simulink model "EV_BMS"  (R2026a)
settings: Solver=VariableStepAuto  StopTime=100
undefined symbols (not defined in the file): battery_builder_rtmsupport, gcbh
libraries: simulink x27, fl_lib x3, nesl_utility x2, EV_BMS_Thermal_lib x1, simulink_extras x1

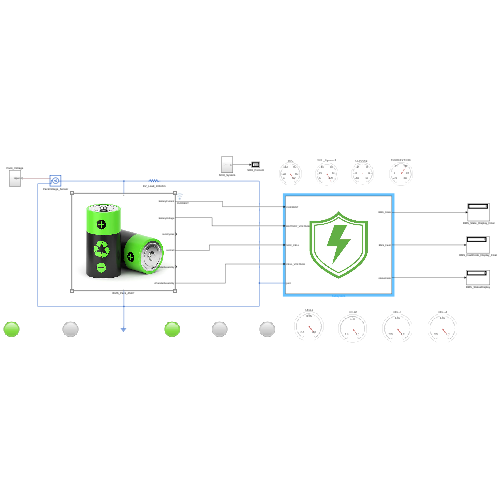
[thumbnail: Simulink's stored preview of the top-level diagram]
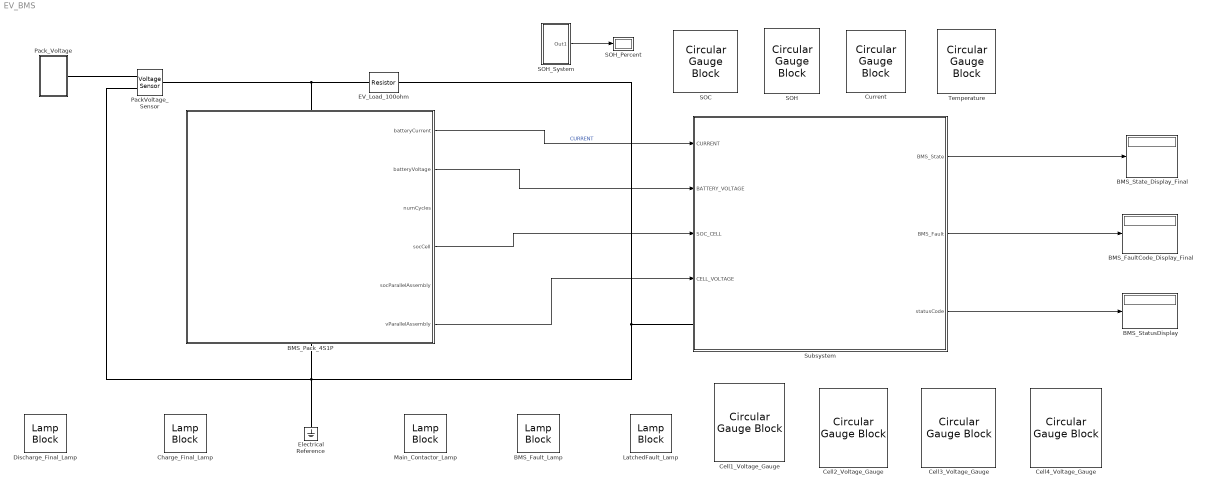
== system EV_BMS ==
  BMS_FaultCode_Display_Final : Display
  BMS_Fault_Lamp : LampBlock  LabelPosition=Hide  DefaultColor=[192.0, 192.0, 192.0]
  BMS_Pack_4S1P : Subsystem  LoadFcn=battery_builder_rtmsupport('loadfcn',gcbh);
      settings: CopyFcn=battery_builder_rtmsupport('copyfcn',gcbh);  PreCopyFcn=battery_builder_rtmsupport('precopyfcn',gcbh);  PreDeleteFcn=battery_builder_rtmsupport('predeletefcn',gcbh);  PortSchema="{\"entries\":[{\"content\":{\"sides\":[{\"content\":{\"connectorIds\":[\"LConn1\"]},\"type\":\"ConnectorPlacement.EquallySpacedRectSide\",\"uuid\":\"f9609fd6-83a3-4776-8a05-b3fc995cf9f2\"},{\"content\":{\"connectorIds\":[\"RConn1\"],\"side\":\"RIGHT\"},\"type\":\"ConnectorPlacement.EquallySpacedRectSide\",\"uuid\":\"cb6b546a-39c6-443d-8083-a29f501cd994\"},{\"content\":{\"side\":\"TOP\"},\"type\":\"ConnectorPlacement.EquallySpacedRectSide\",\"uuid\":\"97627d3a-e8ea-48cc-9b43-c4f6fa748c18\"},{\"content\":{\"connectorIds\":[\"Out1\",\"Out2\",\"Out3\",\"Out4\",\"Out5\",\"Out6\"],\"side\":\"BOTTOM\"},\"type\":\"ConnectorPlacement.EquallySpacedRectSide\",\"uuid\":\"a53582b5-eaea-45ee-b7fe-337964f2a653\"}]},\"type\":\"ConnectorPlacement.EquallySpacedConnector\",\"uuid\":\"342c31db-417c-4e7c-9c09-9d8ea7b34008\"}],\"packageUris\":[\"http://schema.mathworks.com/mf0/Connector/R2020b\"],\"version\":\"1.0\"}"
      mask Display: image('WhatsApp Image 2026-08-24 at 3.32.36 PM (1).jpeg');
  BMS_State_Display_Final : Display
  BMS_StatusDisplay : Display
  Cell1_Voltage_Gauge : CircularGaugeBlock  ScaleMin=2.5  ScaleMax=4.2  FontColor=[0.0, 0.0, 0.0]
  Cell2_Voltage_Gauge : CircularGaugeBlock  ScaleMin=2.5  ScaleMax=4.2  FontColor=[0.0, 0.0, 0.0]
  Cell3_Voltage_Gauge : CircularGaugeBlock  ScaleMin=2.5  ScaleMax=4.2  FontColor=[0.0, 0.0, 0.0]
  Cell4_Voltage_Gauge : CircularGaugeBlock  ScaleMin=2.5  ScaleMax=4.2  FontColor=[0.0, 0.0, 0.0]
  Charge_Final_Lamp : LampBlock  LabelPosition=Hide  DefaultColor=[192.0, 192.0, 192.0]
  Current : CircularGaugeBlock  ScaleMin=-10  ScaleMax=10  FontColor=[0.0, 0.0, 0.0]
  Discharge_Final_Lamp : LampBlock  LabelPosition=Hide  DefaultColor=[192.0, 192.0, 192.0]
  EV_Load_100ohm : fl_lib/Electrical/Electrical Elements/Resistor  R=10 Ohm  i_specify=off  i_priority=None  i=0 A  i_nominal_specify=off  i_nominal_value=1  i_nominal_unit=A  v_specify=off  v_priority=None  v=0 V  v_nominal_specify=off  v_nominal_value=1  v_nominal_unit=V
  Electrical Reference : fl_lib/Electrical/Electrical Elements/Electrical Reference
  LatchedFault_Lamp : LampBlock  LabelPosition=Hide  DefaultColor=[192.0, 192.0, 192.0]
  Main_Contactor_Lamp : LampBlock  LabelPosition=Hide  DefaultColor=[192.0, 192.0, 192.0]
  PackVoltage_Sensor : fl_lib/Electrical/Electrical Sensors/Voltage Sensor
  Pack_Voltage : Subsystem
  SOC : CircularGaugeBlock  FontColor=[0.0, 0.0, 0.0]
  SOH : CircularGaugeBlock  FontColor=[0.0, 0.0, 0.0]
  SOH_Percent : Display
  SOH_System : Subsystem
  Subsystem : Subsystem
      mask Display: image('WhatsApp Image 2026-08-24 at 3.45.53 PM.jpeg');
  Temperature : CircularGaugeBlock  ScaleMin=-20  ScaleMax=60  FontColor=[0.0, 0.0, 0.0]
  wires:
  SOH_System/1(Out1) -> SOH_Percent/1
  BMS_Pack_4S1P/1(batteryCurrent) -> Subsystem/1(CURRENT)  "CURRENT"
  BMS_Pack_4S1P/2(batteryVoltage) -> Subsystem/2(BATTERY_VOLTAGE)
  BMS_Pack_4S1P/4(socCell) -> Subsystem/3(SOC_CELL)
  BMS_Pack_4S1P/6(vParallelAssembly) -> Subsystem/4(CELL_VOLTAGE)
  Subsystem/1(BMS_State) -> BMS_State_Display_Final/1
  Subsystem/2(BMS_Fault) -> BMS_FaultCode_Display_Final/1
  Subsystem/3(statusCode) -> BMS_StatusDisplay/1
  connections:
  PackVoltage_Sensor/RConn2 -- Subsystem/LConn1 -- EV_Load_100ohm/RConn1 -- BMS_Pack_4S1P/RConn1 -- Electrical Reference/LConn1
  EV_Load_100ohm/LConn1 -- BMS_Pack_4S1P/LConn1 -- PackVoltage_Sensor/LConn1
  Pack_Voltage/LConn1 -- PackVoltage_Sensor/RConn1

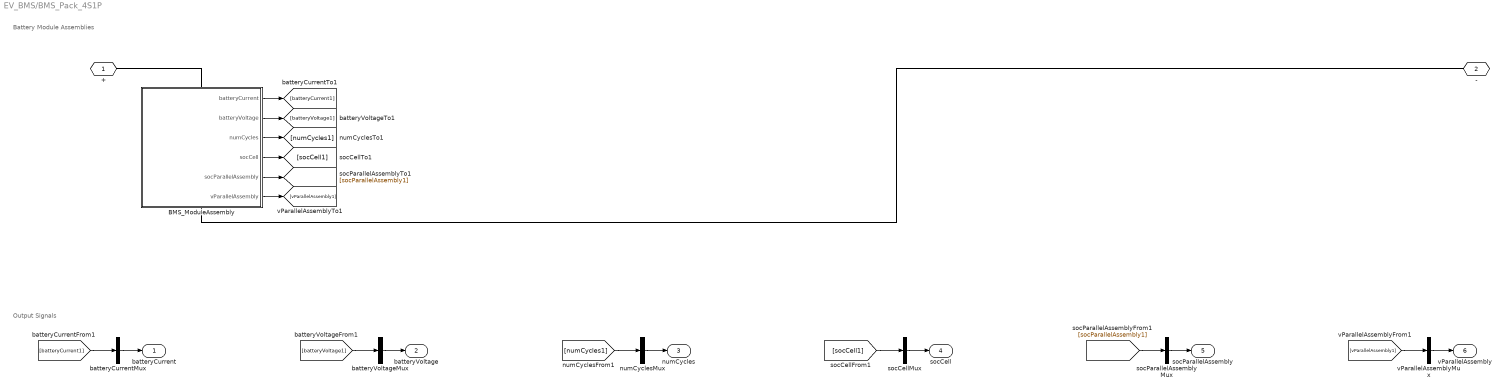
== system EV_BMS/BMS_Pack_4S1P ==
  note: Battery Module Assemblies
  note: Output Signals
  BMS_ModuleAssembly : Subsystem  LoadFcn=battery_builder_rtmsupport('loadfcn',gcbh);
      settings: CopyFcn=battery_builder_rtmsupport('copyfcn',gcbh);  PreCopyFcn=battery_builder_rtmsupport('precopyfcn',gcbh);  PreDeleteFcn=battery_builder_rtmsupport('predeletefcn',gcbh);  PortSchema="{\"entries\":[{\"content\":{\"sides\":[{\"content\":{\"connectorIds\":[\"LConn1\"]},\"type\":\"ConnectorPlacement.EquallySpacedRectSide\",\"uuid\":\"f9609fd6-83a3-4776-8a05-b3fc995cf9f2\"},{\"content\":{\"connectorIds\":[\"RConn1\"],\"side\":\"RIGHT\"},\"type\":\"ConnectorPlacement.EquallySpacedRectSide\",\"uuid\":\"cb6b546a-39c6-443d-8083-a29f501cd994\"},{\"content\":{\"side\":\"TOP\"},\"type\":\"ConnectorPlacement.EquallySpacedRectSide\",\"uuid\":\"97627d3a-e8ea-48cc-9b43-c4f6fa748c18\"},{\"content\":{\"connectorIds\":[\"Out1\",\"Out2\",\"Out3\",\"Out4\",\"Out5\",\"Out6\"],\"side\":\"BOTTOM\"},\"type\":\"ConnectorPlacement.EquallySpacedRectSide\",\"uuid\":\"d854d543-752b-4c93-bd7e-44390da1a379\"}]},\"type\":\"ConnectorPlacement.EquallySpacedConnector\",\"uuid\":\"342c31db-417c-4e7c-9c09-9d8ea7b34008\"}],\"packageUris\":[\"http://schema.mathworks.com/mf0/Connector/R2020b\"],\"version\":\"1.0\"}"
      mask Display: image('moduleAssembly_1.JPG');
  batteryCurrentMux : Mux  Inputs=1
  batteryVoltageMux : Mux  Inputs=1
  numCyclesMux : Mux  Inputs=1
  socCellMux : Mux  Inputs=1
  socParallelAssemblyMux : Mux  Inputs=1
  vParallelAssemblyMux : Mux  Inputs=1
  + : PMIOPort  Side=Left
  - : PMIOPort  Port=2  Side=Right
  batteryCurrent : Outport
  batteryVoltage : Outport  Port=2
  numCycles : Outport  Port=3
  socCell : Outport  Port=4
  socParallelAssembly : Outport  Port=5
  vParallelAssembly : Outport  Port=6
  wires:
  BMS_ModuleAssembly/1(batteryCurrent) -> [batteryCurrent1]
  batteryCurrentMux/1 -> batteryCurrent/1
  [batteryCurrent1] -> batteryCurrentMux/1
  BMS_ModuleAssembly/2(batteryVoltage) -> [batteryVoltage1]
  batteryVoltageMux/1 -> batteryVoltage/1
  [batteryVoltage1] -> batteryVoltageMux/1
  BMS_ModuleAssembly/3(numCycles) -> [numCycles1]
  numCyclesMux/1 -> numCycles/1
  [numCycles1] -> numCyclesMux/1
  BMS_ModuleAssembly/4(socCell) -> [socCell1]
  socCellMux/1 -> socCell/1
  [socCell1] -> socCellMux/1
  BMS_ModuleAssembly/5(socParallelAssembly) -> [socParallelAssembly1]
  socParallelAssemblyMux/1 -> socParallelAssembly/1
  [socParallelAssembly1] -> socParallelAssemblyMux/1
  BMS_ModuleAssembly/6(vParallelAssembly) -> [vParallelAssembly1]
  vParallelAssemblyMux/1 -> vParallelAssembly/1
  [vParallelAssembly1] -> vParallelAssemblyMux/1
  connections:
  BMS_ModuleAssembly/LConn1 -- +/RConn1
  BMS_ModuleAssembly/RConn1 -- -/RConn1

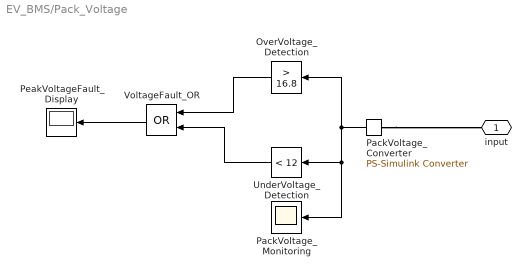
== system EV_BMS/Pack_Voltage ==
  " PackVoltage_Converter" : nesl_utility/PS-Simulink Converter  PhysicalDomain=network_engine_domain  SubClassName=ps_output  LeftPortType=input  RightPortType=output  PseudoPeriodic=off  Frequencies=[]  VectorFormat=inherit  Unit=inherit  AffineConversion=off
  OverVoltage_Detection : simulink/Logic and Bit Operations/Compare To Constant  relop=>  const=16.8  OutDataTypeStr=boolean
  PackVoltage_Monitoring : Scope
      settings: ActiveDisplayYMinimum=16.664557176862598  ActiveDisplayYMaximum=16.709356827128964
  PeakVoltageFault_Display : Display
  UnderVoltage_Detection : simulink/Logic and Bit Operations/Compare To Constant  relop=<  const=12  OutDataTypeStr=boolean
  VoltageFault_OR : Logic  Operator=OR  AllPortsSameDT=off  OutDataTypeStr=boolean
  input : PMIOPort  Side=Left
  wires:
  " PackVoltage_Converter"/1 -> PackVoltage_Monitoring/1, UnderVoltage_Detection/1, OverVoltage_Detection/1
  VoltageFault_OR/1 -> PeakVoltageFault_Display/1
  OverVoltage_Detection/1 -> VoltageFault_OR/1
  UnderVoltage_Detection/1 -> VoltageFault_OR/2
  connections:
  " PackVoltage_Converter"/LConn1 -- input/RConn1

== system EV_BMS/SOH_System ==
  Available_Capacity : Constant  Value=10
  Divide : Product  Inputs=*/
  Gain1 : Gain  Gain=100
  Rated_Capacity : Constant  Value=10
  Out1 : Outport
  wires:
  Rated_Capacity/1 -> Divide/2
  Available_Capacity/1 -> Divide/1
  Divide/1 -> Gain1/1
  Gain1/1 -> Out1/1

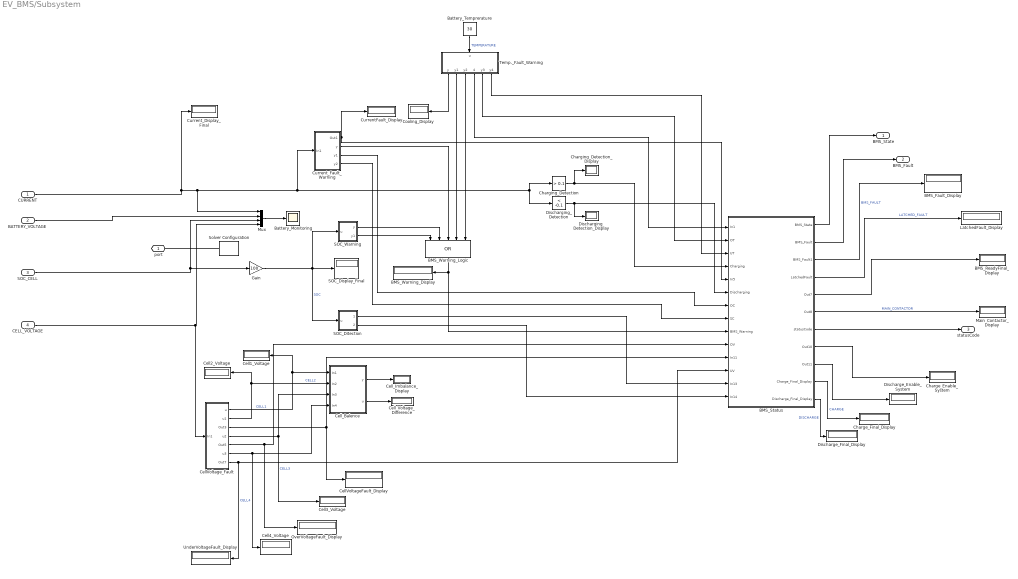
== system EV_BMS/Subsystem ==
  CURRENT : Inport
  BATTERY_VOLTAGE : Inport  Port=2
  SOC_CELL : Inport  Port=3
  CELL_VOLTAGE : Inport  Port=4
  BMS_Fault_Display : Display
  BMS_ReadyFinal_Display : Display
  BMS_Status : Subsystem
  BMS_Warning_Display : Display
  BMS_Warning_Logic : Logic  Operator=OR  Inputs=5  AllPortsSameDT=off  OutDataTypeStr=boolean
  Battery_Monitoring : Scope
      settings: ActiveDisplayYMinimum=-3.3250860487135681  ActiveDisplayYMaximum=5.1404092347440722
  Battery_Temprerature : Constant  Value=30
  Cell1_Voltage : Display
  Cell2_Voltage : Display
  Cell3_Voltage : Display
  Cell4_Voltage : Display
  CellVoltageFault_Display : Display
  CellVoltage_Fault : Subsystem
  Cell_Balence : Subsystem
  Cell_Imbalance_Display : Display
  Cell_Voltage_Difference : Display
  Charge_Enable_System : Display
  Charge_Final_Display : Display
  Charging_Detection : simulink/Logic and Bit Operations/Compare To Constant  relop=>  const=0.1  OutDataTypeStr=boolean
  Charging_Detection_Display : Display
  Cooling_Display : Display
  CurrentFault_Display : Display
  Current_Display_Final : Display
  Current_Fault_Warning : Subsystem
  Discharge_Enable_System : Display
  Discharge_Final_Display : Display
  Discharging_Detection : simulink/Logic and Bit Operations/Compare To Constant  relop=<  const=-0.1  OutDataTypeStr=boolean
  Discharging_Detection_Display : Display
  Gain : Gain  Gain=100
  LatchedFault_Display : Display
  Main_Contactor_Display : Display
  Mux : Mux
  OverVoltageFault_Display : Display
  SOC_Display_Final : Display
  SOC_Ditection : Subsystem
  SOC_Warning : Subsystem
  Solver Configuration : nesl_utility/Solver Configuration  PhysicalDomain=network_engine_domain  SubClassName=solver  LeftPortType=input  RightPortType=generic  Tones=[]  Harmonics=[]  SimulateNoise=off  Profile=off  UseLocalSampling=off  EnableSwitchedLinearOptims=on  FrequencyDomain=off  UseCCode=off  RelTol=0.001  AbsTol=0.001  MinStep=1e-09  ToWorkspace=off  RevertToSquareIcSolve=off  NumHomotopyIterations=100  PhasorMode=off  PhasorModeNumHarmonics=1  ConsistencySolver=NEWTON_XTOL_AFTER_FTOL  CanonicalOrdering=CANONICAL  OptimizeIntermediates=OPTIMIZED  IndexReductionMethod=DerivativeReplacement  DoDC=off  ResidualTolerance=1e-09  ConsistencyTolSource=GLOBAL  ConsistencyAbsTol=0.001  ConsistencyRelTol=0.001  ConsistencyTolFactor=0.001  UseLocalSolver=off  LocalSolverChoice=NE_BACKWARD_EULER_ADVANCER  ResolveIndetEquations=on  FunctionEvalNumThread=1  LocalSolverSampleTime=0.001  DoFixedCost=off  MaxNonlinIter=3  MaxModeIter=2  ComputeImpulses=off  ImpulseIterations=2  LinearAlgebra=auto  LinearAlgebraNumThread=0  EquationFormulation=NE_TIME_EF  DelaysMemoryBudget=1024  AutomaticFiltering=on  FilteringTimeConstant=0.001  PartitionStorageMethod=AS_NEEDED  PartitionMemoryBudget=1024  PartitionMethod=ROBUST  MultibodyUseLocalSolver=off  MultibodyLocalSolverChoice=ODE1  MultibodyLocalSolverSampleTime=0.001
  Temp._Fault_Warning : Subsystem
  UnderVoltageFault_Display : Display
  port : PMIOPort  Side=Left
  BMS_State : Outport
  BMS_Fault : Outport  Port=2
  statusCode : Outport  Port=3
  wires:
  BMS_Status/6(Out8) -> Main_Contactor_Display/1  "MAIN_CONTACTOR"
  Cell_Balence/2(u) -> Cell_Voltage_Difference/1
  BMS_Status/10(Charge_Final_Display) -> Charge_Final_Display/1  "CHARGE"
  BMS_Status/4(LatchedFault) -> LatchedFault_Display/1  "LATCHED_FAULT"
  SOC_Warning/1(y) -> BMS_Warning_Logic/2
  Cell_Balence/1(y) -> Cell_Imbalance_Display/1
  Temp._Fault_Warning/4(Out4) -> BMS_Status/1(In1)
  BMS_Status/3(BMS_Fault1) -> BMS_Fault_Display/1  "BMS_FAULT"
  CellVoltage_Fault/1(u) -> Cell1_Voltage/1, Cell_Balence/1(In1)  "CELL1"
  Current_Fault_Warning/2(y) -> BMS_Warning_Logic/3
  Temp._Fault_Warning/1(y) -> Cooling_Display/1
  SOC_Ditection/1(Out1) -> BMS_Status/13(In13)
  BMS_Status/11(Discharge_Final_Display) -> Discharge_Final_Display/1  "DISCHARGE"
  Temp._Fault_Warning/5(y3) -> BMS_Status/2(OT)
  CellVoltage_Fault/6(u3) -> Cell4_Voltage/1, Cell_Balence/4(In4)  "CELL4"
  Battery_Temprerature/1 -> Temp._Fault_Warning/1(u)  "TEMPERATURE"
  Temp._Fault_Warning/2(y1) -> BMS_Warning_Logic/4
  SOC_Ditection/2(Out2) -> BMS_Status/14(In14)
  Current_Fault_Warning/3(y1) -> BMS_Status/7(OC)
  BMS_Status/2(BMS_Fault) -> BMS_Fault/1
  CellVoltage_Fault/4(u2) -> Cell3_Voltage/1, Cell_Balence/3(In3)  "CELL3"
  Charging_Detection/1 -> Charging_Detection_Display/1, BMS_Status/4(Charging)
  Temp._Fault_Warning/6(y4) -> BMS_Status/3(UT)
  CELL_VOLTAGE/1 -> Mux/4, CellVoltage_Fault/1(In1)
  BMS_Status/5(Out7) -> BMS_ReadyFinal_Display/1
  CURRENT/1 -> Current_Display_Final/1, Charging_Detection/1, Discharging_Detection/1, Current_Fault_Warning/1(In1), Mux/1
  CellVoltage_Fault/3(Out3) -> BMS_Status/11(In11), CellVoltageFault_Display/1
  BMS_Status/1(BMS_State) -> BMS_State/1
  BMS_Warning_Logic/1 -> BMS_Status/9(BMS_Warning), BMS_Warning_Display/1
  Gain/1 -> SOC_Warning/1(u), SOC_Display_Final/1, SOC_Ditection/1(u)  "SOC"
  BATTERY_VOLTAGE/1 -> Mux/2
  BMS_Status/7(statusCode) -> statusCode/1
  Current_Fault_Warning/1(Out1) -> BMS_Status/5(In5), CurrentFault_Display/1
  SOC_CELL/1 -> Mux/3, Gain/1
  Temp._Fault_Warning/3(y2) -> BMS_Warning_Logic/5
  SOC_Warning/2(y1) -> BMS_Warning_Logic/1
  CellVoltage_Fault/5(Out5) -> BMS_Status/10(OV), OverVoltageFault_Display/1
  Current_Fault_Warning/4(y2) -> BMS_Status/8(SC)
  CellVoltage_Fault/7(Out7) -> UnderVoltageFault_Display/1, BMS_Status/12(UV)
  CellVoltage_Fault/2(u1) -> Cell_Balence/2(In2), Cell2_Voltage/1  "CELL2"
  BMS_Status/8(Out10) -> Charge_Enable_System/1
  Mux/1 -> Battery_Monitoring/1
  Discharging_Detection/1 -> BMS_Status/6(Discharging), Discharging_Detection_Display/1
  BMS_Status/9(Out11) -> Discharge_Enable_System/1
  connections:
  Solver Configuration/RConn1 -- port/RConn1

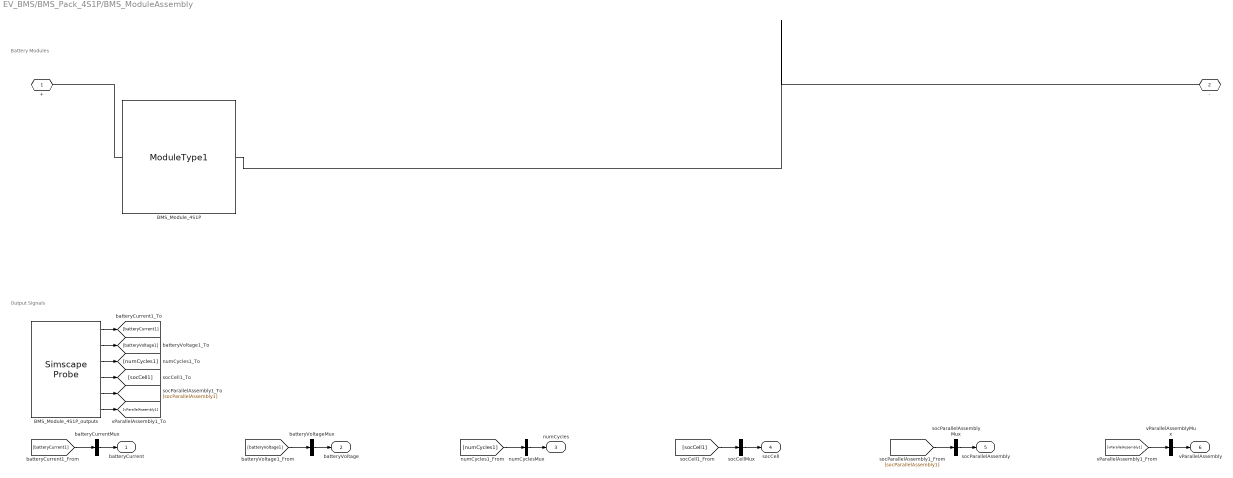
== system EV_BMS/BMS_Pack_4S1P/BMS_ModuleAssembly ==
  note: Output Signals
  note: Battery Modules
  BMS_Module_4S1P : EV_BMS_Thermal_lib/Modules/ModuleType1  BatteryCapacityCell=2.5 A*hr  ExtrapolationMethodCell=simscape.enum.extrapolation.nearest  SOCBreakpointsCell=[0, .1, .25, .5, .75, .9, 1]  TemperatureBreakpointsCell=[278, 293, 313] K  OpenCircuitVoltageThermalCell=[3.49, 3.5, 3.51; 3.55, 3.57, 3.56; 3.62, 3.63, 3.64; 3.71, 3.71, 3.72; 3.91, 3.93, 3.94; 4.07, 4.08, 4.08; 4.19, 4.19, 4.19] V  VoltageRangeCell=[0, inf] V  ResistanceSOCBreakpointsCell=[0, .1, .25, .5, .75, .9, 1]  ResistanceTemperatureBreakpointsCell=[278, 293, 313] K  R0ThermalCell=[.0117, .0085, .009; .011, .0085, .009; .0114, .0087, .0092; .0107, .0082, .0088; .0107, .0083, .0091; .0113, .0085, .0089; .0116, .0085, .0089] Ohm  SimulationTemperatureCell=298.15 K  socCell_specify=off  socCell_priority=High  socCell=1  socCell_nominal_specify=off  socCell_nominal_value=1  socCell_nominal_unit=1  batteryVoltage_specify=off  batteryVoltage_priority=None  batteryVoltage=0 V  batteryVoltage_nominal_specify=off  batteryVoltage_nominal_value=1  batteryVoltage_nominal_unit=V  batteryCurrent_specify=off  batteryCurrent_priority=None  batteryCurrent=0 A  batteryCurrent_nominal_specify=off  batteryCurrent_nominal_value=1  batteryCurrent_nominal_unit=A  numCycles_specify=off  numCycles_priority=High  numCycles=0  numCycles_nominal_specify=off  numCycles_nominal_value=1  numCycles_nominal_unit=1  vParallelAssembly_specify=off  vParallelAssembly_priority=None  vParallelAssembly=repmat(0, 4, 1) V  vParallelAssembly_nominal_specify=off  vParallelAssembly_nominal_value=1  vParallelAssembly_nominal_unit=V  socParallelAssembly_specify=off  socParallelAssembly_priority=None  socParallelAssembly=repmat(1, 4, 1)  socParallelAssembly_nominal_specify=off  socParallelAssembly_nominal_value=1  socParallelAssembly_nominal_unit=1
  BMS_Module_4S1P_outputs : SimscapeProbe  BoundBlock=138  Variables="{\"batteryCurrent\":{\"Probing\":\"ON\"},\"batteryVoltage\":{\"Probing\":\"ON\"},\"numCycles\":{\"Probing\":\"ON\"},\"socCell\":{\"Probing\":\"ON\"},\"socParallelAssembly\":{\"Probing\":\"ON\"},\"vParallelAssembly\":{\"Probing\":\"ON\"}}"
  batteryCurrentMux : Mux  Inputs=1
  batteryVoltageMux : Mux  Inputs=1
  numCyclesMux : Mux  Inputs=1
  socCellMux : Mux  Inputs=1
  socParallelAssemblyMux : Mux  Inputs=1
  vParallelAssemblyMux : Mux  Inputs=1
  + : PMIOPort  Side=Left
  - : PMIOPort  Port=2  Side=Right
  batteryCurrent : Outport
  batteryVoltage : Outport  Port=2
  numCycles : Outport  Port=3
  socCell : Outport  Port=4
  socParallelAssembly : Outport  Port=5
  vParallelAssembly : Outport  Port=6
  wires:
  [vParallelAssembly1] -> vParallelAssemblyMux/1
  vParallelAssemblyMux/1 -> vParallelAssembly/1
  BMS_Module_4S1P_outputs/6 -> [vParallelAssembly1]
  [socParallelAssembly1] -> socParallelAssemblyMux/1
  socParallelAssemblyMux/1 -> socParallelAssembly/1
  BMS_Module_4S1P_outputs/5 -> [socParallelAssembly1]
  [socCell1] -> socCellMux/1
  socCellMux/1 -> socCell/1
  BMS_Module_4S1P_outputs/4 -> [socCell1]
  [numCycles1] -> numCyclesMux/1
  numCyclesMux/1 -> numCycles/1
  BMS_Module_4S1P_outputs/3 -> [numCycles1]
  [batteryVoltage1] -> batteryVoltageMux/1
  batteryVoltageMux/1 -> batteryVoltage/1
  BMS_Module_4S1P_outputs/2 -> [batteryVoltage1]
  [batteryCurrent1] -> batteryCurrentMux/1
  batteryCurrentMux/1 -> batteryCurrent/1
  BMS_Module_4S1P_outputs/1 -> [batteryCurrent1]
  connections:
  BMS_Module_4S1P/RConn1 -- -/RConn1
  BMS_Module_4S1P/LConn1 -- +/RConn1

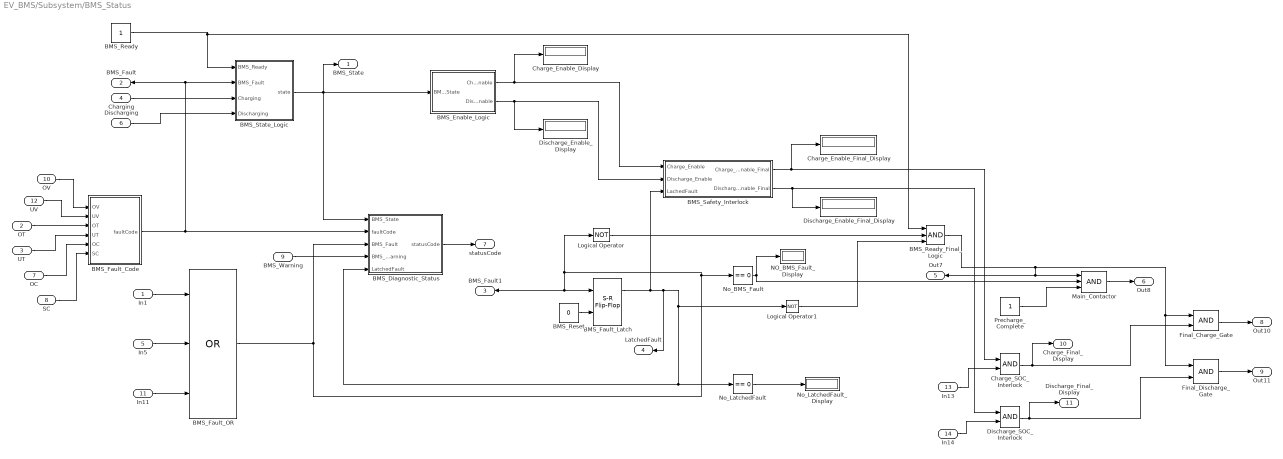
== system EV_BMS/Subsystem/BMS_Status ==
  In1 : Inport
  OT : Inport  Port=2
  UT : Inport  Port=3
  Charging : Inport  Port=4
  In5 : Inport  Port=5
  Discharging : Inport  Port=6
  OC : Inport  Port=7
  SC : Inport  Port=8
  BMS_Warning : Inport  Port=9
  OV : Inport  Port=10
  In11 : Inport  Port=11
  UV : Inport  Port=12
  In13 : Inport  Port=13
  In14 : Inport  Port=14
  BMS_Diagnostic_Status : MATLAB Function  TreatAsAtomicUnit=on
  BMS_Enable_Logic : MATLAB Function  TreatAsAtomicUnit=on
  BMS_Fault_Code : MATLAB Function  TreatAsAtomicUnit=on
  "BMS_Fault_Latch " : simulink_extras/Flip Flops/S-R Flip-Flop  initial_condition=0
  BMS_Fault_OR : Logic  Operator=OR  Inputs=3  AllPortsSameDT=off  OutDataTypeStr=boolean
  BMS_Ready : Constant  OutDataTypeStr=boolean
  BMS_Ready_Final_Logic : Logic  Inputs=3  AllPortsSameDT=off  OutDataTypeStr=boolean
  BMS_Reset : Constant  Value=0  OutDataTypeStr=boolean
  BMS_Safety_Interlock : MATLAB Function  TreatAsAtomicUnit=on
  BMS_State_Logic : MATLAB Function  TreatAsAtomicUnit=on
  Charge_Enable_Display : Display
  Charge_Enable_Final_Display : Display
  Charge_SOC_Interlock : Logic  AllPortsSameDT=off  OutDataTypeStr=boolean
  Discharge_Enable_Display : Display
  Discharge_Enable_Final_Display : Display
  Discharge_SOC_Interlock : Logic  AllPortsSameDT=off  OutDataTypeStr=boolean
  Final_Charge_Gate : Logic  AllPortsSameDT=off  OutDataTypeStr=boolean
  Final_Discharge_Gate : Logic  AllPortsSameDT=off  OutDataTypeStr=boolean
  Logical Operator : Logic  Operator=NOT  AllPortsSameDT=off  OutDataTypeStr=boolean
  Logical Operator1 : Logic  Operator=NOT  AllPortsSameDT=off  OutDataTypeStr=boolean
  Main_Contactor : Logic  Inputs=3  AllPortsSameDT=off  OutDataTypeStr=boolean
  NO_BMS_Fault_Display : Display
  No_BMS_Fault : simulink/Logic and Bit Operations/Compare To Constant  relop===  const=0  OutDataTypeStr=boolean
  No_LatchedFault : simulink/Logic and Bit Operations/Compare To Constant  relop===  const=0  OutDataTypeStr=boolean
  No_LatchedFault_Display : Display
  Precharge_Complete : Constant
  BMS_State : Outport
  BMS_Fault : Outport  Port=2
  BMS_Fault1 : Outport  Port=3
  LatchedFault : Outport  Port=4
  Out7 : Outport  Port=5
  Out8 : Outport  Port=6
  statusCode : Outport  Port=7
  Out10 : Outport  Port=8
  Out11 : Outport  Port=9
  Charge_Final_Display : Outport  Port=10
  Discharge_Final_Display : Outport  Port=11
  wires:
  OT/1 -> BMS_Fault_Code/3(OT)
  Precharge_Complete/1 -> Main_Contactor/3
  Logical Operator1/1 -> BMS_Ready_Final_Logic/3
  Charging/1 -> BMS_State_Logic/3(Charging)
  Charge_SOC_Interlock/1 -> Charge_Final_Display/1, Final_Charge_Gate/2
  BMS_Reset/1 -> "BMS_Fault_Latch "/2
  BMS_Fault_OR/1 -> Logical Operator/1, BMS_Fault1/1, "BMS_Fault_Latch "/1, No_BMS_Fault/1, BMS_Diagnostic_Status/3(BMS_Fault)
  Discharge_SOC_Interlock/1 -> Discharge_Final_Display/1, Final_Discharge_Gate/2
  BMS_Enable_Logic/2(Discharge_Enable) -> BMS_Safety_Interlock/2(Discharge_Enable), Discharge_Enable_Display/1
  UV/1 -> BMS_Fault_Code/2(UV)
  In1/1 -> BMS_Fault_OR/1
  BMS_Ready/1 -> BMS_State_Logic/1(BMS_Ready), BMS_Ready_Final_Logic/1
  Discharging/1 -> BMS_State_Logic/4(Discharging)
  BMS_State_Logic/1(state) -> BMS_Enable_Logic/1(BMS_State), BMS_State/1, BMS_Diagnostic_Status/1(BMS_State)
  No_BMS_Fault/1 -> Main_Contactor/2, NO_BMS_Fault_Display/1
  BMS_Ready_Final_Logic/1 -> Final_Charge_Gate/1, Final_Discharge_Gate/1, Out7/1, Main_Contactor/1
  Final_Charge_Gate/1 -> Out10/1
  In11/1 -> BMS_Fault_OR/3
  UT/1 -> BMS_Fault_Code/4(UT)
  Main_Contactor/1 -> Out8/1
  BMS_Safety_Interlock/2(Discharge_Enable_Final) -> Discharge_Enable_Final_Display/1, Discharge_SOC_Interlock/1
  In13/1 -> Charge_SOC_Interlock/2
  In14/1 -> Discharge_SOC_Interlock/2
  Final_Discharge_Gate/1 -> Out11/1
  BMS_Warning/1 -> BMS_Diagnostic_Status/4(BMS_Warning)
  SC/1 -> BMS_Fault_Code/6(SC)
  BMS_Enable_Logic/1(Chare_Enable) -> BMS_Safety_Interlock/1(Charge_Enable), Charge_Enable_Display/1
  In5/1 -> BMS_Fault_OR/2
  "BMS_Fault_Latch "/1 -> BMS_Diagnostic_Status/5(LatchedFault), No_LatchedFault/1, Logical Operator1/1, LatchedFault/1, BMS_Safety_Interlock/3(LachedFault)
  OC/1 -> BMS_Fault_Code/5(OC)
  OV/1 -> BMS_Fault_Code/1(OV)
  BMS_Safety_Interlock/1(Charge_Enable_Final) -> Charge_Enable_Final_Display/1, Charge_SOC_Interlock/1
  BMS_Diagnostic_Status/1(statusCode) -> statusCode/1
  BMS_Fault_Code/1(faultCode) -> BMS_Fault/1, BMS_State_Logic/2(BMS_Fault), BMS_Diagnostic_Status/2(faultCode)
  No_LatchedFault/1 -> No_LatchedFault_Display/1
  Logical Operator/1 -> BMS_Ready_Final_Logic/2

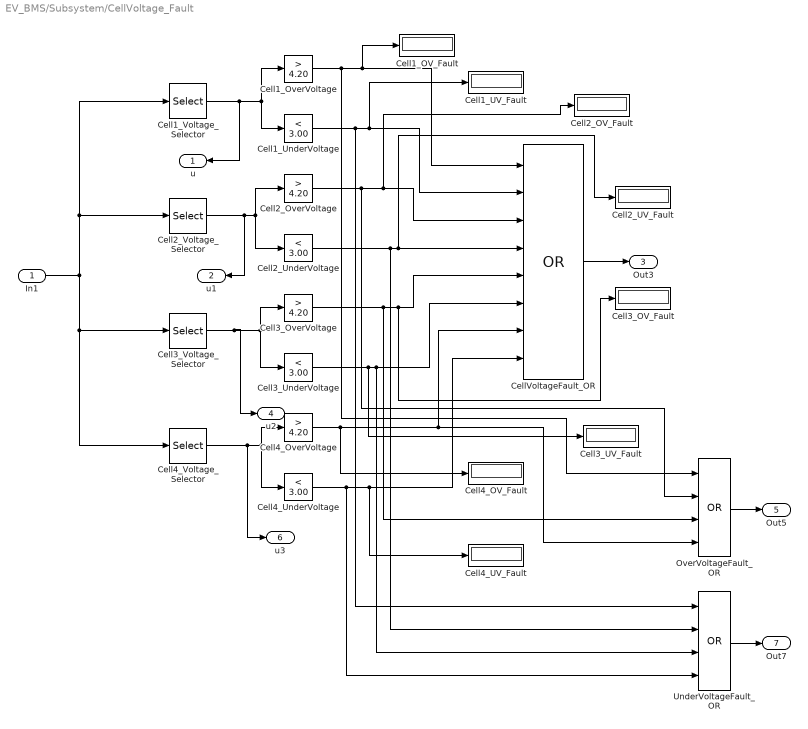
== system EV_BMS/Subsystem/CellVoltage_Fault ==
  In1 : Inport
  Cell1_OV_Fault : Display
  Cell1_OverVoltage : simulink/Logic and Bit Operations/Compare To Constant  relop=>  const=4.20  OutDataTypeStr=boolean
  Cell1_UV_Fault : Display
  Cell1_UnderVoltage : simulink/Logic and Bit Operations/Compare To Constant  relop=<  const=3.00  OutDataTypeStr=boolean
  Cell1_Voltage_Selector : Selector  InputPortWidth=4  IndexOptions=Index vector (dialog)  Indices=[1]  OutputSizes=1
  Cell2_OV_Fault : Display
  Cell2_OverVoltage : simulink/Logic and Bit Operations/Compare To Constant  relop=>  const=4.20  OutDataTypeStr=boolean
  Cell2_UV_Fault : Display
  Cell2_UnderVoltage : simulink/Logic and Bit Operations/Compare To Constant  relop=<  const=3.00  OutDataTypeStr=boolean
  Cell2_Voltage_Selector : Selector  InputPortWidth=4  IndexOptions=Index vector (dialog)  Indices=[2]  OutputSizes=1
  Cell3_OV_Fault : Display
  Cell3_OverVoltage : simulink/Logic and Bit Operations/Compare To Constant  relop=>  const=4.20  OutDataTypeStr=boolean
  Cell3_UV_Fault : Display
  Cell3_UnderVoltage : simulink/Logic and Bit Operations/Compare To Constant  relop=<  const=3.00  OutDataTypeStr=boolean
  Cell3_Voltage_Selector : Selector  InputPortWidth=4  IndexOptions=Index vector (dialog)  Indices=[3]  OutputSizes=1
  Cell4_OV_Fault : Display
  Cell4_OverVoltage : simulink/Logic and Bit Operations/Compare To Constant  relop=>  const=4.20  OutDataTypeStr=boolean
  Cell4_UV_Fault : Display
  Cell4_UnderVoltage : simulink/Logic and Bit Operations/Compare To Constant  relop=<  const=3.00  OutDataTypeStr=boolean
  Cell4_Voltage_Selector : Selector  InputPortWidth=4  IndexOptions=Index vector (dialog)  Indices=[4]  OutputSizes=1
  CellVoltageFault_OR : Logic  Operator=OR  Inputs=8  AllPortsSameDT=off  OutDataTypeStr=boolean
  OverVoltageFault_OR : Logic  Operator=OR  Inputs=4  AllPortsSameDT=off  OutDataTypeStr=boolean
  UnderVoltageFault_OR : Logic  Operator=OR  Inputs=4  AllPortsSameDT=off  OutDataTypeStr=boolean
  u : Outport
  u1 : Outport  Port=2
  Out3 : Outport  Port=3
  u2 : Outport  Port=4
  Out5 : Outport  Port=5
  u3 : Outport  Port=6
  Out7 : Outport  Port=7
  wires:
  Cell1_UnderVoltage/1 -> UnderVoltageFault_OR/1, Cell1_UV_Fault/1, CellVoltageFault_OR/2
  CellVoltageFault_OR/1 -> Out3/1
  Cell4_Voltage_Selector/1 -> u3/1, Cell4_UnderVoltage/1, Cell4_OverVoltage/1
  Cell3_OverVoltage/1 -> OverVoltageFault_OR/3, Cell3_OV_Fault/1, CellVoltageFault_OR/5
  Cell4_UnderVoltage/1 -> UnderVoltageFault_OR/4, Cell4_UV_Fault/1, CellVoltageFault_OR/8
  Cell1_Voltage_Selector/1 -> u/1, Cell1_UnderVoltage/1, Cell1_OverVoltage/1
  Cell2_Voltage_Selector/1 -> u1/1, Cell2_OverVoltage/1, Cell2_UnderVoltage/1
  UnderVoltageFault_OR/1 -> Out7/1
  Cell2_UnderVoltage/1 -> UnderVoltageFault_OR/2, Cell2_UV_Fault/1, CellVoltageFault_OR/4
  OverVoltageFault_OR/1 -> Out5/1
  Cell3_Voltage_Selector/1 -> u2/1, Cell3_UnderVoltage/1, Cell3_OverVoltage/1
  Cell4_OverVoltage/1 -> OverVoltageFault_OR/4, CellVoltageFault_OR/7, Cell4_OV_Fault/1
  In1/1 -> Cell1_Voltage_Selector/1, Cell2_Voltage_Selector/1, Cell4_Voltage_Selector/1, Cell3_Voltage_Selector/1
  Cell2_OverVoltage/1 -> OverVoltageFault_OR/2, CellVoltageFault_OR/3, Cell2_OV_Fault/1
  Cell3_UnderVoltage/1 -> UnderVoltageFault_OR/3, CellVoltageFault_OR/6, Cell3_UV_Fault/1
  Cell1_OverVoltage/1 -> OverVoltageFault_OR/1, Cell1_OV_Fault/1, CellVoltageFault_OR/1

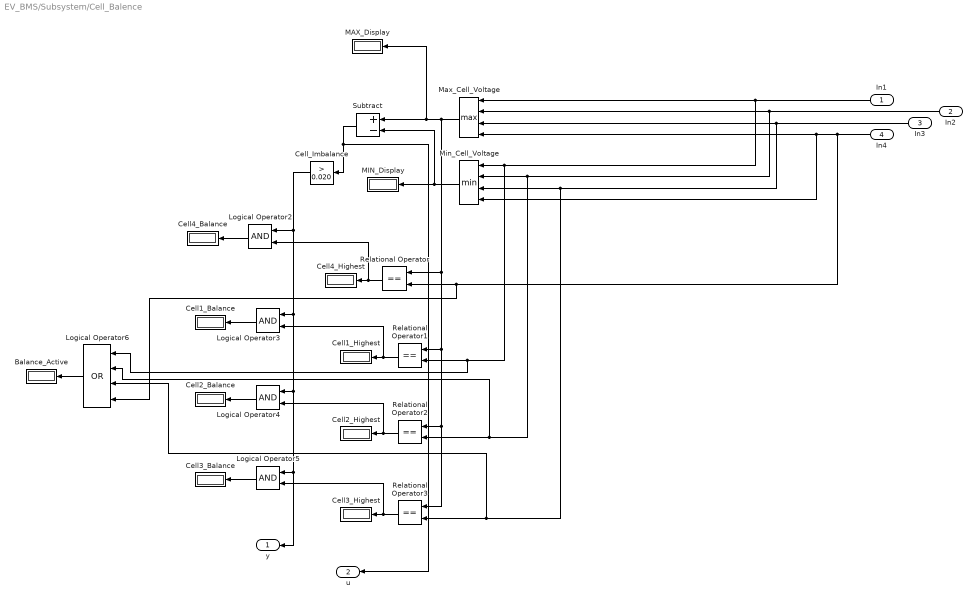
== system EV_BMS/Subsystem/Cell_Balence ==
  In1 : Inport
  In2 : Inport  Port=2
  In3 : Inport  Port=3
  In4 : Inport  Port=4
  Balance_Active : Display
  Cell1_Balance : Display
  "Cell1_Highest " : Display
  Cell2_Balance : Display
  "Cell2_Highest " : Display
  Cell3_Balance : Display
  "Cell3_Highest " : Display
  Cell4_Balance : Display
  "Cell4_Highest " : Display
  Cell_Imbalance : simulink/Logic and Bit Operations/Compare To Constant  relop=>  const=0.020  OutDataTypeStr=boolean
  Logical Operator{2..5} (4 alike) : Logic  AllPortsSameDT=off  OutDataTypeStr=boolean
  Logical Operator6 : Logic  Operator=OR  Inputs=4  AllPortsSameDT=off  OutDataTypeStr=boolean
  MAX_Display : Display
  MIN_Display : Display
  Max_Cell_Voltage : MinMax  Function=max  Inputs=4
  Min_Cell_Voltage : MinMax  Inputs=4
  Relational Operator{,1..3} (4 alike) : RelationalOperator  Operator===  OutDataTypeStr=boolean  RndMeth=Simplest  InputSameDT=off
  Subtract : Sum  Inputs=+-
  y : Outport
  u : Outport  Port=2
  wires:
  Logical Operator6/1 -> Balance_Active/1
  Logical Operator4/1 -> Cell2_Balance/1
  Subtract/1 -> u/1, Cell_Imbalance/1
  Logical Operator3/1 -> Cell1_Balance/1
  Cell_Imbalance/1 -> y/1, Logical Operator5/1, Logical Operator4/1, Logical Operator3/1, Logical Operator2/1
  Relational Operator2/1 -> Logical Operator4/2, "Cell2_Highest "/1
  Relational Operator1/1 -> Logical Operator3/2, "Cell1_Highest "/1
  In3/1 -> Logical Operator6/3, Relational Operator3/2, Min_Cell_Voltage/3, Max_Cell_Voltage/3
  Relational Operator3/1 -> Logical Operator5/2, "Cell3_Highest "/1
  In2/1 -> Max_Cell_Voltage/2, Logical Operator6/2, Relational Operator2/2, Min_Cell_Voltage/2
  Max_Cell_Voltage/1 -> Relational Operator3/1, Relational Operator2/1, Relational Operator1/1, Relational Operator/1, MAX_Display/1, Subtract/1
  Logical Operator2/1 -> Cell4_Balance/1
  Logical Operator5/1 -> Cell3_Balance/1
  In1/1 -> Logical Operator6/1, Relational Operator1/2, Min_Cell_Voltage/1, Max_Cell_Voltage/1
  Min_Cell_Voltage/1 -> Subtract/2, MIN_Display/1
  In4/1 -> Logical Operator6/4, Relational Operator/2, Min_Cell_Voltage/4, Max_Cell_Voltage/4
  Relational Operator/1 -> Logical Operator2/2, "Cell4_Highest "/1

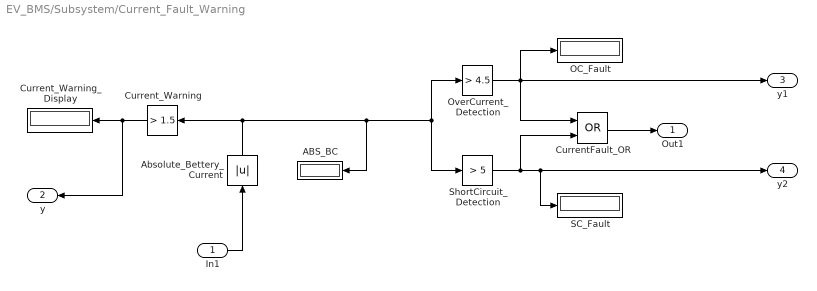
== system EV_BMS/Subsystem/Current_Fault_Warning ==
  In1 : Inport
  ABS_BC : Display
  Absolute_Bettery_Current : Abs  SaturateOnIntegerOverflow=off
  CurrentFault_OR : Logic  Operator=OR  AllPortsSameDT=off  OutDataTypeStr=boolean
  Current_Warning : simulink/Logic and Bit Operations/Compare To Constant  relop=>  const=1.5  OutDataTypeStr=boolean
  Current_Warning_Display : Display
  OC_Fault : Display
  OverCurrent_Detection : simulink/Logic and Bit Operations/Compare To Constant  relop=>  const=4.5  OutDataTypeStr=boolean
  SC_Fault : Display
  ShortCircuit_Detection : simulink/Logic and Bit Operations/Compare To Constant  relop=>  const=5  OutDataTypeStr=boolean
  Out1 : Outport
  y : Outport  Port=2
  y1 : Outport  Port=3
  y2 : Outport  Port=4
  wires:
  CurrentFault_OR/1 -> Out1/1
  Absolute_Bettery_Current/1 -> Current_Warning/1, ShortCircuit_Detection/1, OverCurrent_Detection/1, ABS_BC/1
  ShortCircuit_Detection/1 -> SC_Fault/1, y2/1, CurrentFault_OR/2
  OverCurrent_Detection/1 -> CurrentFault_OR/1, y1/1, OC_Fault/1
  In1/1 -> Absolute_Bettery_Current/1
  Current_Warning/1 -> y/1, Current_Warning_Display/1

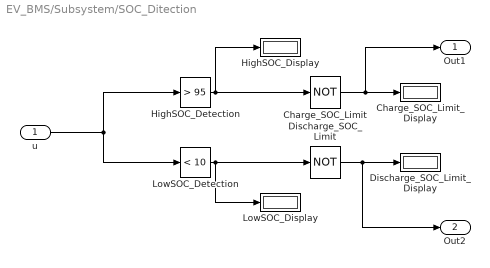
== system EV_BMS/Subsystem/SOC_Ditection ==
  u : Inport
  Charge_SOC_Limit : Logic  Operator=NOT  AllPortsSameDT=off  OutDataTypeStr=boolean
  Charge_SOC_Limit_Display : Display
  Discharge_SOC_Limit : Logic  Operator=NOT  AllPortsSameDT=off  OutDataTypeStr=boolean
  Discharge_SOC_Limit_Display : Display
  HighSOC_Detection : simulink/Logic and Bit Operations/Compare To Constant  relop=>  const=95  OutDataTypeStr=boolean
  HighSOC_Display : Display
  LowSOC_Detection : simulink/Logic and Bit Operations/Compare To Constant  relop=<  const=10  OutDataTypeStr=boolean
  LowSOC_Display : Display
  Out1 : Outport
  Out2 : Outport  Port=2
  wires:
  HighSOC_Detection/1 -> Charge_SOC_Limit/1, HighSOC_Display/1
  Charge_SOC_Limit/1 -> Out1/1, Charge_SOC_Limit_Display/1
  LowSOC_Detection/1 -> Discharge_SOC_Limit/1, LowSOC_Display/1
  u/1 -> LowSOC_Detection/1, HighSOC_Detection/1
  Discharge_SOC_Limit/1 -> Discharge_SOC_Limit_Display/1, Out2/1

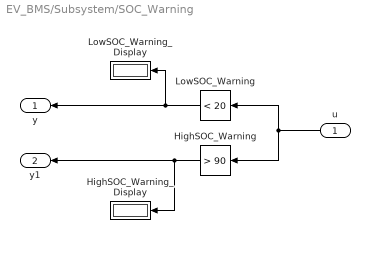
== system EV_BMS/Subsystem/SOC_Warning ==
  u : Inport
  HighSOC_Warning : simulink/Logic and Bit Operations/Compare To Constant  relop=>  const=90  OutDataTypeStr=boolean
  HighSOC_Warning_Display : Display
  LowSOC_Warning : simulink/Logic and Bit Operations/Compare To Constant  relop=<  const=20  OutDataTypeStr=boolean
  LowSOC_Warning_Display : Display
  y : Outport
  y1 : Outport  Port=2
  wires:
  HighSOC_Warning/1 -> y1/1, HighSOC_Warning_Display/1
  LowSOC_Warning/1 -> y/1, LowSOC_Warning_Display/1
  u/1 -> LowSOC_Warning/1, HighSOC_Warning/1

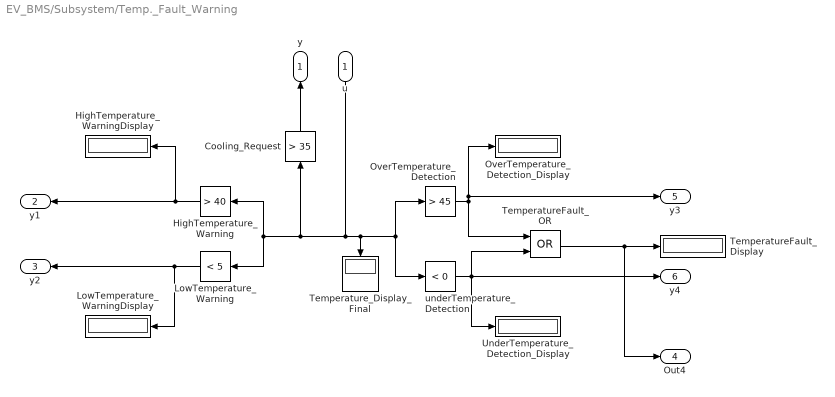
== system EV_BMS/Subsystem/Temp._Fault_Warning ==
  u : Inport
  Cooling_Request : simulink/Logic and Bit Operations/Compare To Constant  relop=>  const=35  OutDataTypeStr=boolean
  HighTemperature_Warning : simulink/Logic and Bit Operations/Compare To Constant  relop=>  const=40  OutDataTypeStr=boolean
  HighTemperature_WarningDisplay : Display
  LowTemperature_Warning : simulink/Logic and Bit Operations/Compare To Constant  relop=<  const=5  OutDataTypeStr=boolean
  LowTemperature_WarningDisplay : Display
  OverTemperature_Detection : simulink/Logic and Bit Operations/Compare To Constant  relop=>  const=45  OutDataTypeStr=boolean
  OverTemperature_Detection_Display : Display
  TemperatureFault_Display : Display
  TemperatureFault_OR : Logic  Operator=OR  AllPortsSameDT=off  OutDataTypeStr=boolean
  Temperature_Display_Final : Display
  UnderTemperature_Detection_Display : Display
  underTemperature_Detection : simulink/Logic and Bit Operations/Compare To Constant  relop=<  const=0  OutDataTypeStr=boolean
  y : Outport
  y1 : Outport  Port=2
  y2 : Outport  Port=3
  Out4 : Outport  Port=4
  y3 : Outport  Port=5
  y4 : Outport  Port=6
  wires:
  HighTemperature_Warning/1 -> y1/1, HighTemperature_WarningDisplay/1
  OverTemperature_Detection/1 -> OverTemperature_Detection_Display/1, y3/1, TemperatureFault_OR/1
  LowTemperature_Warning/1 -> LowTemperature_WarningDisplay/1, y2/1
  Cooling_Request/1 -> y/1
  underTemperature_Detection/1 -> y4/1, TemperatureFault_OR/2, UnderTemperature_Detection_Display/1
  TemperatureFault_OR/1 -> Out4/1, TemperatureFault_Display/1
  u/1 -> Temperature_Display_Final/1, underTemperature_Detection/1, OverTemperature_Detection/1, Cooling_Request/1, LowTemperature_Warning/1, HighTemperature_Warning/1

== matlab function EV_BMS/Subsystem/BMS_Status/BMS_State_Logic ==
  data: BMS_Ready input; BMS_Fault input; state output; Charging input; Discharging input
function state = BMS_State_Logic(BMS_Ready,BMS_Fault,Charging,Discharging)

%State code
%0 = INIT
%1 = Normal/IDLE
%2 = CHARGING
%3 = DISCHARGING
%4 = FAULT
%5 = SHUTDOWN

state = 0; %Default:INIT

if ~BMS_Ready
    state = 0; %INIT
elseif BMS_Fault
    state = 4; %FAULT
elseif Charging
    state = 2; %Charging
elseif Discharging
    state = 3; %Discharging
else 
    state = 1; %Normal/IDLE
end

== matlab function EV_BMS/Subsystem/BMS_Status/BMS_Fault_Code ==
  data: OV input; faultCode output; UV input; OT input; UT input; OC input; SC input
function faultCode = BMS_Fault_Code(OV,UV,OT,UT,OC,SC)

faultCode = 0; 

if SC
    faultCode = 6;
elseif OC 
    faultCode = 5;
elseif UT
    faultCode = 4;
elseif OT
    faultCode = 3;
elseif UV
    faultCode = 2;
elseif OV
    faultCode = 1;
end

== matlab function EV_BMS/Subsystem/BMS_Status/BMS_Enable_Logic ==
  data: Chare_Enable output; Discharge_Enable output; BMS_State input
function [Chare_Enable,Discharge_Enable] = BMS_Enable_Logic(BMS_State)

Chare_Enable = false;
Discharge_Enable = false;

if BMS_State == 1 % Normal/IDLE
    Chare_Enable = true;
    Discharge_Enable = true;
elseif BMS_State == 2 % Charging
    Chare_Enable = true;
elseif BMS_State == 3 % Discharging
    Discharge_Enable = true;
else % INIT/Fault/Shurdown
    Chare_Enable = false;
    Discharge_Enable = false;
end

== matlab function EV_BMS/Subsystem/BMS_Status/BMS_Safety_Interlock ==
  data: Charge_Enable input; Charge_Enable_Final output; Discharge_Enable input; LachedFault input; Discharge_Enable_Final output
function [Charge_Enable_Final,Discharge_Enable_Final] = BMS_Safety_Interlock(Charge_Enable,Discharge_Enable,LachedFault)

if LachedFault
    Charge_Enable_Final = false;
    Discharge_Enable_Final = false;
else
    Charge_Enable_Final = Charge_Enable;
    Discharge_Enable_Final = Discharge_Enable;
end

== matlab function EV_BMS/Subsystem/BMS_Status/BMS_Diagnostic_Status ==
  data: BMS_State input; statusCode output; faultCode input; BMS_Fault input; BMS_Warning input; LatchedFault input
function statusCode = BMS_Diagnostic_Status(BMS_State,faultCode,BMS_Fault,BMS_Warning,LatchedFault)

%Diagnostic status codes
%0 = SystemOK
%1 = Warning
%2 = Active Fault
%3 = Latched Fault
%4 = INIT
%5 = SHUTDOWN

if LatchedFault
    statusCode = 3;
elseif BMS_Fault
    statusCode = 2;
elseif BMS_State == 0
    statusCode = 4;
elseif BMS_State == 5
    statusCode = 5;
elseif BMS_Warning
    statusCode = 1;
else
    statusCode = 0;
end
